simulink model "StarshipSystemModel"  (R2025b)
settings: Solver=VariableStepAuto  StartTime=0.0  StopTime=10.0  RelTol=1e-3
model workspace (MAT data in the model file):
  ActiveGNCMode : Simulink.Bus (value not decoded)
  AerodynamicControlCommand : Simulink.Bus (value not decoded)
  AerodynamicLoad : Simulink.Bus (value not decoded)
  AggregatedStream : Simulink.Bus (value not decoded)
  AllocatedEffectorDemand : Simulink.Bus (value not decoded)
  AttitudeControlDemand : Simulink.Bus (value not decoded)
  AttitudeGuidanceCommand : Simulink.Bus (value not decoded)
  AttitudeRateState : Simulink.Bus (value not decoded)
  AutogenousPressurantGas : Simulink.ConnectionBus (value not decoded)
  CandidateFaultIndication : Simulink.Bus (value not decoded)
  CombustionGasFeed : Simulink.ConnectionBus (value not decoded)
  CommandPathHealth : Simulink.Bus (value not decoded)
  ControlMode : Simulink.ValueType (value not decoded)
  DownlinkSignal : Simulink.Bus (value not decoded)
  ElectricalPower : Simulink.ConnectionBus (value not decoded)
  EngineTelemetry : Simulink.Bus (value not decoded)
  ExecutionContext : Simulink.Bus (value not decoded)
  FaultDiagnosisResult : Simulink.Bus (value not decoded)
  GNCDataContext : Simulink.Bus (value not decoded)
  GNCHealthState : Simulink.Bus (value not decoded)
  GNCStateEstimate : Simulink.Bus (value not decoded)
  GimbalAngle : Simulink.ValueType (value not decoded)
  GimbalMotion : Simulink.ConnectionBus (value not decoded)
  GroundCheckoutLink : Simulink.Bus (value not decoded)
  GroundPressurantSupply : Simulink.ConnectionBus (value not decoded)
  GuidanceConstraints : Simulink.Bus (value not decoded)
  GuidanceMode : Simulink.ValueType (value not decoded)
  LinkHealth : Simulink.Bus (value not decoded)
  LiquidPropellantFeed : Simulink.ConnectionBus (value not decoded)
  MechanicalMotion : Simulink.ConnectionBus (value not decoded)
  MechanismPosition : Simulink.Bus (value not decoded)
  ModeTransitionContext : Simulink.Bus (value not decoded)
  NavigationAidingData : Simulink.Bus (value not decoded)
  NavigationEstimate : Simulink.Bus (value not decoded)
  NavigationHealthStatus : Simulink.Bus (value not decoded)
  NavigationMeasurementSet : Simulink.Bus (value not decoded)
  PercentThrottle : Simulink.ValueType (value not decoded)
  PneumaticActuationGas : Simulink.ConnectionBus (value not decoded)
  PowerConversionStatus : Simulink.Bus (value not decoded)
  PowerDistributionStatus : Simulink.Bus (value not decoded)
  PowerHealthStatus : Simulink.Bus (value not decoded)
  PowerManagementCommand : Simulink.Bus (value not decoded)
  PowerStorageStatus : Simulink.Bus (value not decoded)
  ProtectedThermalState : Simulink.Bus (value not decoded)
  ProtectionIsolationStatus : Simulink.Bus (value not decoded)
  PurgeGasSupply : Simulink.ConnectionBus (value not decoded)
  RCSPulseCommand : Simulink.Bus (value not decoded)
  RCSTelemetry : Simulink.Bus (value not decoded)
  RFFeed : Simulink.ConnectionBus (value not decoded)
  RecoveryMechanismCommand : Simulink.Bus (value not decoded)
  RollThrottleBias : Simulink.ValueType (value not decoded)
  SafetyOverride : Simulink.ValueType (value not decoded)
  SafetyStateStatus : Simulink.Bus (value not decoded)
  ShapedControlDemand : Simulink.Bus (value not decoded)
  SpinStartIgniterGas : Simulink.ConnectionBus (value not decoded)
  StageMechanicalBoundary : Simulink.ConnectionBus (value not decoded)
  StructuralLoad : Simulink.ConnectionBus (value not decoded)
  StructureHealthStatus : Simulink.Bus (value not decoded)
  SubsystemHealthEvidence : Simulink.Bus (value not decoded)
  SubsystemStatusTelemetry : Simulink.Bus (value not decoded)
  TankTelemetry : Simulink.Bus (value not decoded)
  ThermalMonitoringCommand : Simulink.Bus (value not decoded)
  ThermalNetwork : Simulink.ConnectionBus (value not decoded)
  ThrustLoad : Simulink.ConnectionBus (value not decoded)
  TrajectoryGuidanceCommand : Simulink.Bus (value not decoded)
  TrajectoryReference : Simulink.Bus (value not decoded)
  TranslationalControlDemand : Simulink.Bus (value not decoded)
  TranslationalState : Simulink.Bus (value not decoded)
  UplinkSignal : Simulink.Bus (value not decoded)
  ValidatedControlDemand : Simulink.Bus (value not decoded)
  ValveCommand : Simulink.ValueType (value not decoded)
  VehicleStructureState : Simulink.Bus (value not decoded)
  VerifiedCommand : Simulink.Bus (value not decoded)
  VideoStream : Simulink.Bus (value not decoded)
undefined symbols (not defined in the file): ACR, ACT, ASM, ATM, BCR, BDQ, BDR, BDX, BEC, BFC, BHV, BIP, BLM, BNZ, BPI, BPR, BPV, BRX, BSM, BTA, BTP, BVC, BVE, BVV, CAA, CAM, CAS, CAT, CLM, COM, CRS, CTL, CTR, DAQ, ESC, EXT, FCR, FDB, FDE, FEX, FHI, FHM, FIC, FIS, FMG, FSC, GAP, GCM, GMD, GNC, GND, GPH, GTR, HDN, HIA, HSI, IF, INT, LOC, NAI ... (+45)
(part 5 of 8)

== system StarshipSystemModel/Starship/Safety & Fault Management /Fault Diagnosis & Isolation ==
  Bus Element In1 : Inport  PortName=IF-FDE-FCR-01
  Fault Correlation & Reasoning : Subsystem
      settings: PortSchema="{\"entries\":[{\"content\":{\"headerSize\":26,\"margin\":15,\"minimumSpacing\":25,\"sides\":[{\"content\":{\"connectorIds\":[\"In1\"]},\"type\":\"ConnectorPlacement.EquallySpacedRectSide\",\"uuid\":\"c1b9b7ae-a5d1-4a08-a561-f06fbe6dc300\"},{\"content\":{\"connectorIds\":[\"Out1\"],\"side\":\"RIGHT\"},\"type\":\"ConnectorPlacement.EquallySpacedRectSide\",\"uuid\":\"af8a3603-108a-44dc-af3d-660c23f2553a\"},{\"content\":{\"side\":\"TOP\"},\"type\":\"ConnectorPlacement.EquallySpacedRectSide\",\"uuid\":\"59101f68-40fe-4ccb-9258-ad0f93699a98\"}]},\"type\":\"ConnectorPlacement.EquallySpacedConnector\",\"uuid\":\"683df2e7-6d18-4135-a0d1-7e7a3e3475d2\"}],\"packageUris\":[\"http://schema.mathworks.com/mf0/Connector/R2020b\"],\"version\":\"1.0\"}"
  Fault Identification & Classification : Subsystem
      settings: PortSchema="{\"entries\":[{\"content\":{\"headerSize\":26,\"margin\":15,\"minimumSpacing\":25,\"sides\":[{\"content\":{\"connectorIds\":[\"In1\"]},\"type\":\"ConnectorPlacement.EquallySpacedRectSide\",\"uuid\":\"c1b9b7ae-a5d1-4a08-a561-f06fbe6dc300\"},{\"content\":{\"connectorIds\":[\"Out1\"],\"side\":\"RIGHT\"},\"type\":\"ConnectorPlacement.EquallySpacedRectSide\",\"uuid\":\"af8a3603-108a-44dc-af3d-660c23f2553a\"},{\"content\":{\"side\":\"TOP\"},\"type\":\"ConnectorPlacement.EquallySpacedRectSide\",\"uuid\":\"59101f68-40fe-4ccb-9258-ad0f93699a98\"}]},\"type\":\"ConnectorPlacement.EquallySpacedConnector\",\"uuid\":\"683df2e7-6d18-4135-a0d1-7e7a3e3475d2\"}],\"packageUris\":[\"http://schema.mathworks.com/mf0/Connector/R2020b\"],\"version\":\"1.0\"}"
  Fault Isolation : Subsystem
      settings: PortSchema="{\"entries\":[{\"content\":{\"headerSize\":26,\"margin\":15,\"minimumSpacing\":25,\"sides\":[{\"content\":{\"connectorIds\":[\"In1\"]},\"type\":\"ConnectorPlacement.EquallySpacedRectSide\",\"uuid\":\"c1b9b7ae-a5d1-4a08-a561-f06fbe6dc300\"},{\"content\":{\"connectorIds\":[\"Out1\"],\"side\":\"RIGHT\"},\"type\":\"ConnectorPlacement.EquallySpacedRectSide\",\"uuid\":\"af8a3603-108a-44dc-af3d-660c23f2553a\"},{\"content\":{\"side\":\"TOP\"},\"type\":\"ConnectorPlacement.EquallySpacedRectSide\",\"uuid\":\"59101f68-40fe-4ccb-9258-ad0f93699a98\"}]},\"type\":\"ConnectorPlacement.EquallySpacedConnector\",\"uuid\":\"683df2e7-6d18-4135-a0d1-7e7a3e3475d2\"}],\"packageUris\":[\"http://schema.mathworks.com/mf0/Connector/R2020b\"],\"version\":\"1.0\"}"
  Bus Element Out1 : Outport  PortName=IF-FIC-SEA-01
  wires:
  Fault Isolation/1(IF-FIS-FIC-01) -> Fault Identification & Classification/1(IF-FIS-FIC-01)
  Bus Element In1/1 -> Fault Correlation & Reasoning/1(IF-FDE-FCR-01)
  Fault Correlation & Reasoning/1(IF-FCR-FIS-01) -> Fault Isolation/1(IF-FCR-FIS-01)
  Fault Identification & Classification/1(IF-FIC-SEA-01) -> Bus Element Out1/1

== system StarshipSystemModel/Starship/Safety & Fault Management /Fault Management & Response Logic ==
  Bus Element In1 : Inport  PortName=IF-FIC-SEA-01
  Protective Action Coordination : Subsystem
      settings: PortSchema="{\"entries\":[{\"content\":{\"headerSize\":26,\"margin\":15,\"minimumSpacing\":25,\"sides\":[{\"content\":{\"connectorIds\":[\"In1\"]},\"type\":\"ConnectorPlacement.EquallySpacedRectSide\",\"uuid\":\"c1b9b7ae-a5d1-4a08-a561-f06fbe6dc300\"},{\"content\":{\"connectorIds\":[\"Out1\",\"Out2\",\"Out3\"],\"side\":\"RIGHT\"},\"type\":\"ConnectorPlacement.EquallySpacedRectSide\",\"uuid\":\"af8a3603-108a-44dc-af3d-660c23f2553a\"},{\"content\":{\"side\":\"TOP\"},\"type\":\"ConnectorPlacement.EquallySpacedRectSide\",\"uuid\":\"59101f68-40fe-4ccb-9258-ad0f93699a98\"}]},\"type\":\"ConnectorPlacement.EquallySpacedConnector\",\"uuid\":\"683df2e7-6d18-4135-a0d1-7e7a3e3475d2\"}],\"packageUris\":[\"http://schema.mathworks.com/mf0/Connector/R2020b\"],\"version\":\"1.0\"}"
  Response Selection Logic : Subsystem
      settings: PortSchema="{\"entries\":[{\"content\":{\"headerSize\":26,\"margin\":15,\"minimumSpacing\":25,\"sides\":[{\"content\":{\"connectorIds\":[\"In1\"]},\"type\":\"ConnectorPlacement.EquallySpacedRectSide\",\"uuid\":\"c1b9b7ae-a5d1-4a08-a561-f06fbe6dc300\"},{\"content\":{\"connectorIds\":[\"Out1\"],\"side\":\"RIGHT\"},\"type\":\"ConnectorPlacement.EquallySpacedRectSide\",\"uuid\":\"af8a3603-108a-44dc-af3d-660c23f2553a\"},{\"content\":{\"side\":\"TOP\"},\"type\":\"ConnectorPlacement.EquallySpacedRectSide\",\"uuid\":\"59101f68-40fe-4ccb-9258-ad0f93699a98\"}]},\"type\":\"ConnectorPlacement.EquallySpacedConnector\",\"uuid\":\"683df2e7-6d18-4135-a0d1-7e7a3e3475d2\"}],\"packageUris\":[\"http://schema.mathworks.com/mf0/Connector/R2020b\"],\"version\":\"1.0\"}"
  Severity & Consequence Assessment : Subsystem
      settings: PortSchema="{\"entries\":[{\"content\":{\"headerSize\":26,\"margin\":15,\"minimumSpacing\":25,\"sides\":[{\"content\":{\"connectorIds\":[\"In1\"]},\"type\":\"ConnectorPlacement.EquallySpacedRectSide\",\"uuid\":\"c1b9b7ae-a5d1-4a08-a561-f06fbe6dc300\"},{\"content\":{\"connectorIds\":[\"Out1\"],\"side\":\"RIGHT\"},\"type\":\"ConnectorPlacement.EquallySpacedRectSide\",\"uuid\":\"af8a3603-108a-44dc-af3d-660c23f2553a\"},{\"content\":{\"side\":\"TOP\"},\"type\":\"ConnectorPlacement.EquallySpacedRectSide\",\"uuid\":\"59101f68-40fe-4ccb-9258-ad0f93699a98\"}]},\"type\":\"ConnectorPlacement.EquallySpacedConnector\",\"uuid\":\"683df2e7-6d18-4135-a0d1-7e7a3e3475d2\"}],\"packageUris\":[\"http://schema.mathworks.com/mf0/Connector/R2020b\"],\"version\":\"1.0\"}"
  Bus Element Out1 : Outport  PortName=IF-SAF-BEC-01
  Bus Element Out2 : Outport  Port=2  PortName=IF-SAF-SEC-01
  Bus Element Out3 : Outport  Port=3  PortName=IF-PAC-RCO-01
  wires:
  Protective Action Coordination/2(IF-SAF-SEC-01) -> Bus Element Out2/1
  Response Selection Logic/1(IF-RSL-PAC-01) -> Protective Action Coordination/1(IF-RSL-PAC-01)
  Bus Element In1/1 -> Severity & Consequence Assessment/1(IF-FIC-SEA-01)
  Severity & Consequence Assessment/1(IF-SEA-RSL-01) -> Response Selection Logic/1(IF-SEA-RSL-01)
  Protective Action Coordination/3(IF-PAC-RCO-01) -> Bus Element Out3/1
  Protective Action Coordination/1(IF-SAF-BEC-01) -> Bus Element Out1/1

== system StarshipSystemModel/Starship/Safety & Fault Management /Health Monitoring & Fault Detection ==
  Bus Element In11 : Inport  PortName=IF-RSM-SAF-01
  Bus Element In10 : Inport  Port=2  PortName=IF-INT-SAF-01
  Bus Element In9 : Inport  Port=3  PortName=IF-POS-SAF-01
  Bus Element In8 : Inport  Port=4  PortName=IF-TMS-SAF-01
  Bus Element In7 : Inport  Port=5  PortName=IF-FHM-SAF-01
  Bus Element In1 : Inport  Port=6  PortName=IF-BEC-SAF-01
  Bus Element In2 : Inport  Port=7  PortName=IF-SEC-SAF-01
  Bus Element In3 : Inport  Port=8  PortName=IF-RCT-SAF-01
  Bus Element In4 : Inport  Port=9  PortName=IF-BPR-SAF-01
  Bus Element In5 : Inport  Port=10  PortName=IF-SPR-SAF-01
  Bus Element In6 : Inport  Port=11  PortName=IF-PMM-SAF-01
  Bus Element In12 : Inport  Port=12  PortName=IF-BLM-SAF-01
  Bus Element In13 : Inport  Port=13  PortName=IF-SLM-SAF-01
  Bus Element In14 : Inport  Port=14  PortName=IF-ESC-HIA-01
  Fault Detection Engine : Subsystem
      settings: PortSchema="{\"entries\":[{\"content\":{\"headerSize\":26,\"margin\":15,\"minimumSpacing\":25,\"sides\":[{\"content\":{\"connectorIds\":[\"In1\"]},\"type\":\"ConnectorPlacement.EquallySpacedRectSide\",\"uuid\":\"c1b9b7ae-a5d1-4a08-a561-f06fbe6dc300\"},{\"content\":{\"connectorIds\":[\"Out1\"],\"side\":\"RIGHT\"},\"type\":\"ConnectorPlacement.EquallySpacedRectSide\",\"uuid\":\"af8a3603-108a-44dc-af3d-660c23f2553a\"},{\"content\":{\"side\":\"TOP\"},\"type\":\"ConnectorPlacement.EquallySpacedRectSide\",\"uuid\":\"59101f68-40fe-4ccb-9258-ad0f93699a98\"}]},\"type\":\"ConnectorPlacement.EquallySpacedConnector\",\"uuid\":\"683df2e7-6d18-4135-a0d1-7e7a3e3475d2\"}],\"packageUris\":[\"http://schema.mathworks.com/mf0/Connector/R2020b\"],\"version\":\"1.0\"}"
  Health Information Aggregation : Subsystem
      settings: PortSchema="{\"entries\":[{\"content\":{\"headerSize\":26,\"margin\":15,\"minimumSpacing\":25,\"sides\":[{\"content\":{\"connectorIds\":[\"In1\",\"In2\",\"In3\",\"In4\",\"In5\",\"In6\",\"In7\",\"In8\",\"In9\",\"In10\",\"In11\",\"In12\",\"In13\",\"In14\"]},\"type\":\"ConnectorPlacement.EquallySpacedRectSide\",\"uuid\":\"c1b9b7ae-a5d1-4a08-a561-f06fbe6dc300\"},{\"content\":{\"connectorIds\":[\"Out1\"],\"side\":\"RIGHT\"},\"type\":\"ConnectorPlacement.EquallySpacedRectSide\",\"uuid\":\"af8a3603-108a-44dc-af3d-660c23f2553a\"},{\"content\":{\"side\":\"TOP\"},\"type\":\"ConnectorPlacement.EquallySpacedRectSide\",\"uuid\":\"59101f68-40fe-4ccb-9258-ad0f93699a98\"}]},\"type\":\"ConnectorPlacement.EquallySpacedConnector\",\"uuid\":\"683df2e7-6d18-4135-a0d1-7e7a3e3475d2\"}],\"packageUris\":[\"http://schema.mathworks.com/mf0/Connector/R2020b\"],\"version\":\"1.0\"}"
  Validity & Integrity Evaluation : Subsystem
      settings: PortSchema="{\"entries\":[{\"content\":{\"headerSize\":26,\"margin\":15,\"minimumSpacing\":25,\"sides\":[{\"content\":{\"connectorIds\":[\"In1\"]},\"type\":\"ConnectorPlacement.EquallySpacedRectSide\",\"uuid\":\"c1b9b7ae-a5d1-4a08-a561-f06fbe6dc300\"},{\"content\":{\"connectorIds\":[\"Out1\"],\"side\":\"RIGHT\"},\"type\":\"ConnectorPlacement.EquallySpacedRectSide\",\"uuid\":\"af8a3603-108a-44dc-af3d-660c23f2553a\"},{\"content\":{\"side\":\"TOP\"},\"type\":\"ConnectorPlacement.EquallySpacedRectSide\",\"uuid\":\"59101f68-40fe-4ccb-9258-ad0f93699a98\"}]},\"type\":\"ConnectorPlacement.EquallySpacedConnector\",\"uuid\":\"683df2e7-6d18-4135-a0d1-7e7a3e3475d2\"}],\"packageUris\":[\"http://schema.mathworks.com/mf0/Connector/R2020b\"],\"version\":\"1.0\"}"
  Bus Element Out1 : Outport  PortName=IF-FDE-FCR-01
  wires:
  Bus Element In11/1 -> Health Information Aggregation/1(IF-RSM-SAF-01)
  Bus Element In10/1 -> Health Information Aggregation/2(IF-INT-SAF-01)
  Bus Element In3/1 -> Health Information Aggregation/8(IF-RCT-SAF-01)
  Bus Element In2/1 -> Health Information Aggregation/7(IF-SEC-SAF-01)
  Bus Element In1/1 -> Health Information Aggregation/6(IF-BEC-SAF-01)
  Bus Element In9/1 -> Health Information Aggregation/3(IF-POS-SAF-01)
  Bus Element In7/1 -> Health Information Aggregation/5(IF-FHM-SAF-01)
  Bus Element In8/1 -> Health Information Aggregation/4(IF-TMS-SAF-01)
  Bus Element In4/1 -> Health Information Aggregation/9(IF-BPR-SAF-01)
  Bus Element In5/1 -> Health Information Aggregation/10(IF-SPR-SAF-01)
  Bus Element In6/1 -> Health Information Aggregation/11(IF-PMM-SAF-01)
  Validity & Integrity Evaluation/1(IF-VIE-FDE-01) -> Fault Detection Engine/1(IF-VIE-FDE-01)
  Bus Element In12/1 -> Health Information Aggregation/12(IF-BLM-SAF-01)
  Bus Element In13/1 -> Health Information Aggregation/13(IF-SLM-SAF-01)
  Bus Element In14/1 -> Health Information Aggregation/14(IF-ESC-HIA-01)
  Health Information Aggregation/1(IF-HIA-VIE-01) -> Validity & Integrity Evaluation/1(IF-HIA-VIE-01)
  Fault Detection Engine/1(IF-FDE-FCR-01) -> Bus Element Out1/1

== system StarshipSystemModel/Starship/Safety & Fault Management /Recovery & Reconfiguration Management ==
  Bus Element In1 : Inport  PortName=IF-PAC-RCO-01
  Reconfiguration Coordinator : Subsystem
      settings: PortSchema="{\"entries\":[{\"content\":{\"headerSize\":26,\"margin\":15,\"minimumSpacing\":25,\"sides\":[{\"content\":{\"connectorIds\":[\"In1\"]},\"type\":\"ConnectorPlacement.EquallySpacedRectSide\",\"uuid\":\"c1b9b7ae-a5d1-4a08-a561-f06fbe6dc300\"},{\"content\":{\"connectorIds\":[\"Out1\"],\"side\":\"RIGHT\"},\"type\":\"ConnectorPlacement.EquallySpacedRectSide\",\"uuid\":\"af8a3603-108a-44dc-af3d-660c23f2553a\"},{\"content\":{\"side\":\"TOP\"},\"type\":\"ConnectorPlacement.EquallySpacedRectSide\",\"uuid\":\"59101f68-40fe-4ccb-9258-ad0f93699a98\"}]},\"type\":\"ConnectorPlacement.EquallySpacedConnector\",\"uuid\":\"683df2e7-6d18-4135-a0d1-7e7a3e3475d2\"}],\"packageUris\":[\"http://schema.mathworks.com/mf0/Connector/R2020b\"],\"version\":\"1.0\"}"
  Recovery Sequence Executor : Subsystem
      settings: PortSchema="{\"entries\":[{\"content\":{\"headerSize\":26,\"margin\":15,\"minimumSpacing\":25,\"sides\":[{\"content\":{\"connectorIds\":[\"In1\"]},\"type\":\"ConnectorPlacement.EquallySpacedRectSide\",\"uuid\":\"c1b9b7ae-a5d1-4a08-a561-f06fbe6dc300\"},{\"content\":{\"connectorIds\":[\"Out1\",\"Out2\"],\"side\":\"RIGHT\"},\"type\":\"ConnectorPlacement.EquallySpacedRectSide\",\"uuid\":\"af8a3603-108a-44dc-af3d-660c23f2553a\"},{\"content\":{\"side\":\"TOP\"},\"type\":\"ConnectorPlacement.EquallySpacedRectSide\",\"uuid\":\"59101f68-40fe-4ccb-9258-ad0f93699a98\"}]},\"type\":\"ConnectorPlacement.EquallySpacedConnector\",\"uuid\":\"683df2e7-6d18-4135-a0d1-7e7a3e3475d2\"}],\"packageUris\":[\"http://schema.mathworks.com/mf0/Connector/R2020b\"],\"version\":\"1.0\"}"
  Recovery Verification : Subsystem
      settings: PortSchema="{\"entries\":[{\"content\":{\"headerSize\":26,\"margin\":15,\"minimumSpacing\":25,\"sides\":[{\"content\":{\"connectorIds\":[\"In1\"]},\"type\":\"ConnectorPlacement.EquallySpacedRectSide\",\"uuid\":\"c1b9b7ae-a5d1-4a08-a561-f06fbe6dc300\"},{\"content\":{\"connectorIds\":[\"Out1\"],\"side\":\"RIGHT\"},\"type\":\"ConnectorPlacement.EquallySpacedRectSide\",\"uuid\":\"af8a3603-108a-44dc-af3d-660c23f2553a\"},{\"content\":{\"side\":\"TOP\"},\"type\":\"ConnectorPlacement.EquallySpacedRectSide\",\"uuid\":\"59101f68-40fe-4ccb-9258-ad0f93699a98\"}]},\"type\":\"ConnectorPlacement.EquallySpacedConnector\",\"uuid\":\"683df2e7-6d18-4135-a0d1-7e7a3e3475d2\"}],\"packageUris\":[\"http://schema.mathworks.com/mf0/Connector/R2020b\"],\"version\":\"1.0\"}"
  Bus Element Out1 : Outport  PortName=IF-SAF-RSM-01
  Bus Element Out2 : Outport  Port=2  PortName=IF-RVF-SSM-01
  wires:
  Recovery Sequence Executor/2(IF-RSE-RVF-01) -> Recovery Verification/1(IF-RSE-RVF-01)
  Bus Element In1/1 -> Reconfiguration Coordinator/1(IF-PAC-RCO-01)
  Reconfiguration Coordinator/1(IF-RCO-RSE-01) -> Recovery Sequence Executor/1(IF-RCO-RSE-01)
  Recovery Sequence Executor/1(IF-SAF-RSM-01) -> Bus Element Out1/1
  Recovery Verification/1(IF-RVF-SSM-01) -> Bus Element Out2/1

== system StarshipSystemModel/Starship/Safety & Fault Management /Safety State & Flight-Safety Management ==
  Bus Element In3 : Inport  PortName=IF-RVF-SSM-01
  Bus Element In1 : Inport  Port=2  PortName=IF-BCR-SAF-01
  Bus Element In2 : Inport  Port=3  PortName=IF-SCR-SAF-01
  Escalation & Containment Status : Subsystem
      settings: PortSchema="{\"entries\":[{\"content\":{\"headerSize\":26,\"margin\":15,\"minimumSpacing\":25,\"sides\":[{\"content\":{\"connectorIds\":[\"In1\"]},\"type\":\"ConnectorPlacement.EquallySpacedRectSide\",\"uuid\":\"c1b9b7ae-a5d1-4a08-a561-f06fbe6dc300\"},{\"content\":{\"connectorIds\":[\"Out2\",\"Out1\",\"Out3\"],\"side\":\"RIGHT\"},\"type\":\"ConnectorPlacement.EquallySpacedRectSide\",\"uuid\":\"af8a3603-108a-44dc-af3d-660c23f2553a\"},{\"content\":{\"side\":\"TOP\"},\"type\":\"ConnectorPlacement.EquallySpacedRectSide\",\"uuid\":\"59101f68-40fe-4ccb-9258-ad0f93699a98\"},{\"content\":{\"side\":\"BOTTOM\"},\"type\":\"ConnectorPlacement.EquallySpacedRectSide\",\"uuid\":\"baebb347-8adb-49bd-9e46-495e8e474d7d\"}]},\"type\":\"ConnectorPlacement.EquallySpacedConnector\",\"uuid\":\"683df2e7-6d18-4135-a0d1-7e7a3e3475d2\"}],\"packageUris\":[\"http://schema.mathworks.com/mf0/Connector/R2020b\"],\"version\":\"1.0\"}"
  Flight-Safety Coordination : Subsystem
      settings: PortSchema="{\"entries\":[{\"content\":{\"headerSize\":26,\"margin\":15,\"minimumSpacing\":25,\"sides\":[{\"content\":{\"connectorIds\":[\"In1\",\"In2\",\"In3\"]},\"type\":\"ConnectorPlacement.EquallySpacedRectSide\",\"uuid\":\"c1b9b7ae-a5d1-4a08-a561-f06fbe6dc300\"},{\"content\":{\"connectorIds\":[\"Out1\"],\"side\":\"RIGHT\"},\"type\":\"ConnectorPlacement.EquallySpacedRectSide\",\"uuid\":\"af8a3603-108a-44dc-af3d-660c23f2553a\"},{\"content\":{\"side\":\"TOP\"},\"type\":\"ConnectorPlacement.EquallySpacedRectSide\",\"uuid\":\"59101f68-40fe-4ccb-9258-ad0f93699a98\"}]},\"type\":\"ConnectorPlacement.EquallySpacedConnector\",\"uuid\":\"683df2e7-6d18-4135-a0d1-7e7a3e3475d2\"}],\"packageUris\":[\"http://schema.mathworks.com/mf0/Connector/R2020b\"],\"version\":\"1.0\"}"
  Safety State Manager : Subsystem
      settings: PortSchema="{\"entries\":[{\"content\":{\"headerSize\":26,\"margin\":15,\"minimumSpacing\":25,\"sides\":[{\"content\":{\"connectorIds\":[\"In1\"]},\"type\":\"ConnectorPlacement.EquallySpacedRectSide\",\"uuid\":\"c1b9b7ae-a5d1-4a08-a561-f06fbe6dc300\"},{\"content\":{\"connectorIds\":[\"Out1\",\"Out2\"],\"side\":\"RIGHT\"},\"type\":\"ConnectorPlacement.EquallySpacedRectSide\",\"uuid\":\"af8a3603-108a-44dc-af3d-660c23f2553a\"},{\"content\":{\"side\":\"TOP\"},\"type\":\"ConnectorPlacement.EquallySpacedRectSide\",\"uuid\":\"59101f68-40fe-4ccb-9258-ad0f93699a98\"}]},\"type\":\"ConnectorPlacement.EquallySpacedConnector\",\"uuid\":\"683df2e7-6d18-4135-a0d1-7e7a3e3475d2\"}],\"packageUris\":[\"http://schema.mathworks.com/mf0/Connector/R2020b\"],\"version\":\"1.0\"}"
  Bus Element Out2 : Outport  PortName=IF-SAF-BTA-01
  Bus Element Out3 : Outport  Port=2  PortName=IF-SAF-STA-01
  Bus Element Out1 : Outport  Port=3  PortName=IF-SAF-FHM-01
  Bus Element Out4 : Outport  Port=4  PortName=IF-ESC-HIA-01
  wires:
  Flight-Safety Coordination/1(IF-FSC-ESC-01) -> Escalation & Containment Status/1(IF-FSC-ESC-01)
  Bus Element In3/1 -> Safety State Manager/1(IF-RVF-SSM-01)
  Safety State Manager/2(IF-SSM-FSC-01) -> Flight-Safety Coordination/3(IF-SSM-FSC-01)
  Escalation & Containment Status/2(IF-SAF-BTA-01) -> Bus Element Out2/1
  Bus Element In1/1 -> Flight-Safety Coordination/1(IF-BCR-SAF-01)
  Bus Element In2/1 -> Flight-Safety Coordination/2(IF-SCR-SAF-01)
  Safety State Manager/1(IF-SAF-FHM-01) -> Bus Element Out1/1
  Escalation & Containment Status/1(IF-SAF-STA-01) -> Bus Element Out3/1
  Escalation & Containment Status/3(IF-ESC-HIA-01) -> Bus Element Out4/1

== system StarshipSystemModel/Starship/Structure and Mechanisms/Aerodynamic Control Mechanisms ==
  Bus Element In1 : Inport  PortName=IF-GNC-ACT-01
  Bus Element In2 : Inport  Port=2  PortName=IF-ATM-SUR-01
  Actuator : Subsystem
      settings: PortSchema="{\"entries\":[{\"content\":{\"headerSize\":26,\"margin\":15,\"minimumSpacing\":25,\"sides\":[{\"content\":{\"connectorIds\":[\"In1\",\"In2\",\"LConn1\"]},\"type\":\"ConnectorPlacement.EquallySpacedRectSide\",\"uuid\":\"23792f18-2863-4199-9730-8799d4a474a5\"},{\"content\":{\"connectorIds\":[\"RConn1\"],\"side\":\"RIGHT\"},\"type\":\"ConnectorPlacement.EquallySpacedRectSide\",\"uuid\":\"c8cda51b-7b41-45d2-a922-70343296893f\"},{\"content\":{\"side\":\"TOP\"},\"type\":\"ConnectorPlacement.EquallySpacedRectSide\",\"uuid\":\"3580f4a1-1924-4d7f-ad03-70e3a97c03ce\"}]},\"type\":\"ConnectorPlacement.EquallySpacedConnector\",\"uuid\":\"f1529067-176f-4d7b-82ef-d3d6162373fd\"}],\"packageUris\":[\"http://schema.mathworks.com/mf0/Connector/R2020b\"],\"version\":\"1.0\"}"
  Hinge / linkage : Subsystem
      settings: PortSchema="{\"entries\":[{\"content\":{\"headerSize\":26,\"margin\":15,\"minimumSpacing\":25,\"sides\":[{\"content\":{\"connectorIds\":[\"LConn1\",\"LConn2\"]},\"type\":\"ConnectorPlacement.EquallySpacedRectSide\",\"uuid\":\"23792f18-2863-4199-9730-8799d4a474a5\"},{\"content\":{\"connectorIds\":[\"RConn1\",\"RConn2\"],\"side\":\"RIGHT\"},\"type\":\"ConnectorPlacement.EquallySpacedRectSide\",\"uuid\":\"c8cda51b-7b41-45d2-a922-70343296893f\"},{\"content\":{\"side\":\"TOP\"},\"type\":\"ConnectorPlacement.EquallySpacedRectSide\",\"uuid\":\"3580f4a1-1924-4d7f-ad03-70e3a97c03ce\"}]},\"type\":\"ConnectorPlacement.EquallySpacedConnector\",\"uuid\":\"f1529067-176f-4d7b-82ef-d3d6162373fd\"}],\"packageUris\":[\"http://schema.mathworks.com/mf0/Connector/R2020b\"],\"version\":\"1.0\"}"
  Position / health : Subsystem
      settings: PortSchema="{\"entries\":[{\"content\":{\"headerSize\":26,\"margin\":15,\"minimumSpacing\":25,\"sides\":[{\"content\":{},\"type\":\"ConnectorPlacement.EquallySpacedRectSide\",\"uuid\":\"23792f18-2863-4199-9730-8799d4a474a5\"},{\"content\":{\"connectorIds\":[\"Out1\",\"Out2\",\"Out3\"],\"side\":\"RIGHT\"},\"type\":\"ConnectorPlacement.EquallySpacedRectSide\",\"uuid\":\"c8cda51b-7b41-45d2-a922-70343296893f\"},{\"content\":{\"side\":\"TOP\"},\"type\":\"ConnectorPlacement.EquallySpacedRectSide\",\"uuid\":\"3580f4a1-1924-4d7f-ad03-70e3a97c03ce\"}]},\"type\":\"ConnectorPlacement.EquallySpacedConnector\",\"uuid\":\"f1529067-176f-4d7b-82ef-d3d6162373fd\"}],\"packageUris\":[\"http://schema.mathworks.com/mf0/Connector/R2020b\"],\"version\":\"1.0\"}"
  Surface / fin / flap : Subsystem
      settings: PortSchema="{\"entries\":[{\"content\":{\"headerSize\":26,\"margin\":15,\"minimumSpacing\":25,\"sides\":[{\"content\":{\"connectorIds\":[\"In1\",\"LConn1\"]},\"type\":\"ConnectorPlacement.EquallySpacedRectSide\",\"uuid\":\"23792f18-2863-4199-9730-8799d4a474a5\"},{\"content\":{\"connectorIds\":[\"RConn1\"],\"side\":\"RIGHT\"},\"type\":\"ConnectorPlacement.EquallySpacedRectSide\",\"uuid\":\"c8cda51b-7b41-45d2-a922-70343296893f\"},{\"content\":{\"side\":\"TOP\"},\"type\":\"ConnectorPlacement.EquallySpacedRectSide\",\"uuid\":\"3580f4a1-1924-4d7f-ad03-70e3a97c03ce\"}]},\"type\":\"ConnectorPlacement.EquallySpacedConnector\",\"uuid\":\"f1529067-176f-4d7b-82ef-d3d6162373fd\"}],\"packageUris\":[\"http://schema.mathworks.com/mf0/Connector/R2020b\"],\"version\":\"1.0\"}"
  IF-HNG-INT-01 : PMIOPort  Side=Right
  IF-PWR-STR-01 : PMIOPort  Port=2  Side=Left  ConnectionType=Bus: ElectricalPower
  Bus Element Out1 : Outport  PortName=IF-POS-GNC-01
  Bus Element Out2 : Outport  Port=2  PortName=IF-POS-SAF-01
  wires:
  Position / health/1(IF-POS-GNC-01) -> Bus Element Out1/1
  Position / health/2(IF-POS-ACT-01) -> Actuator/2(IF-POS-ACT-01)
  Bus Element In1/1 -> Actuator/1(IF-GNC-ACT-01)
  Bus Element In2/1 -> Surface / fin / flap/1(IF-ATM-SUR-01)
  Position / health/3(IF-POS-SAF-01) -> Bus Element Out2/1
  connections:
  Hinge / linkage/RConn2 -- IF-HNG-INT-01/RConn1
  Actuator/RConn1 -- Hinge / linkage/LConn2
  Hinge / linkage/RConn1 -- Surface / fin / flap/LConn1
  Surface / fin / flap/RConn1 -- Hinge / linkage/LConn1
  IF-PWR-STR-01/RConn1 -- Actuator/LConn1

== system StarshipSystemModel/Starship/Structure and Mechanisms/Primary Load-Bearing Airframe ==
  " Load-transfer structure" : Subsystem
      settings: PortSchema="{\"entries\":[{\"content\":{\"headerSize\":26,\"margin\":15,\"minimumSpacing\":25,\"sides\":[{\"content\":{\"connectorIds\":[\"LConn1\",\"LConn2\"]},\"type\":\"ConnectorPlacement.EquallySpacedRectSide\",\"uuid\":\"23792f18-2863-4199-9730-8799d4a474a5\"},{\"content\":{\"connectorIds\":[\"RConn1\"],\"side\":\"RIGHT\"},\"type\":\"ConnectorPlacement.EquallySpacedRectSide\",\"uuid\":\"c8cda51b-7b41-45d2-a922-70343296893f\"},{\"content\":{\"side\":\"TOP\"},\"type\":\"ConnectorPlacement.EquallySpacedRectSide\",\"uuid\":\"3580f4a1-1924-4d7f-ad03-70e3a97c03ce\"}]},\"type\":\"ConnectorPlacement.EquallySpacedConnector\",\"uuid\":\"f1529067-176f-4d7b-82ef-d3d6162373fd\"}],\"packageUris\":[\"http://schema.mathworks.com/mf0/Connector/R2020b\"],\"version\":\"1.0\"}"
  Local interface structure : Subsystem
      settings: PortSchema="{\"entries\":[{\"content\":{\"headerSize\":26,\"margin\":15,\"minimumSpacing\":25,\"sides\":[{\"content\":{\"connectorIds\":[\"LConn1\",\"LConn2\",\"LConn3\"]},\"type\":\"ConnectorPlacement.EquallySpacedRectSide\",\"uuid\":\"23792f18-2863-4199-9730-8799d4a474a5\"},{\"content\":{\"connectorIds\":[\"Out1\",\"Out2\",\"Out3\",\"RConn1\"],\"side\":\"RIGHT\"},\"type\":\"ConnectorPlacement.EquallySpacedRectSide\",\"uuid\":\"c8cda51b-7b41-45d2-a922-70343296893f\"},{\"content\":{\"side\":\"TOP\"},\"type\":\"ConnectorPlacement.EquallySpacedRectSide\",\"uuid\":\"3580f4a1-1924-4d7f-ad03-70e3a97c03ce\"}]},\"type\":\"ConnectorPlacement.EquallySpacedConnector\",\"uuid\":\"f1529067-176f-4d7b-82ef-d3d6162373fd\"}],\"packageUris\":[\"http://schema.mathworks.com/mf0/Connector/R2020b\"],\"version\":\"1.0\"}"
  Primary pressure/shell : Subsystem
      settings: PortSchema="{\"entries\":[{\"content\":{\"headerSize\":26,\"margin\":15,\"minimumSpacing\":25,\"sides\":[{\"content\":{\"connectorIds\":[\"RConn2\",\"RConn1\",\"LConn1\",\"LConn2\",\"LConn3\",\"LConn4\",\"LConn5\"]},\"type\":\"ConnectorPlacement.EquallySpacedRectSide\",\"uuid\":\"23792f18-2863-4199-9730-8799d4a474a5\"},{\"content\":{\"connectorIds\":[\"RConn3\"],\"side\":\"RIGHT\"},\"type\":\"ConnectorPlacement.EquallySpacedRectSide\",\"uuid\":\"c8cda51b-7b41-45d2-a922-70343296893f\"},{\"content\":{\"side\":\"TOP\"},\"type\":\"ConnectorPlacement.EquallySpacedRectSide\",\"uuid\":\"3580f4a1-1924-4d7f-ad03-70e3a97c03ce\"}]},\"type\":\"ConnectorPlacement.EquallySpacedConnector\",\"uuid\":\"f1529067-176f-4d7b-82ef-d3d6162373fd\"}],\"packageUris\":[\"http://schema.mathworks.com/mf0/Connector/R2020b\"],\"version\":\"1.0\"}"
  IF-TLI-LDT-01 : PMIOPort  Side=Right
  IF-BOT-PRS-01 : PMIOPort  Port=2  Side=Right  ConnectionType=Bus: StructuralLoad
  IF-SOT-PRS-01 : PMIOPort  Port=3  Side=Right  ConnectionType=Bus: StructuralLoad
  IF-TBI-PRS-01 : PMIOPort  Port=4  Side=Left  ConnectionType=Bus: ThermalNetwork
  IF-BTP-PRS-01 : PMIOPort  Port=5  Side=Left  ConnectionType=Bus: ThermalNetwork
  IF-STP-PRS-01 : PMIOPort  Port=6  Side=Left  ConnectionType=Bus: ThermalNetwork
  IF-HNG-INT-01 : PMIOPort  Port=7  Side=Left
  IF-SLS-LDT-01 : PMIOPort  Port=8  Side=Left
  IF-RLI-PRS-01 : PMIOPort  Port=9  Side=Left
  Bus Element Out1 : Outport  PortName=IF-INT-STA-01
  Bus Element Out2 : Outport  Port=2  PortName=IF-INT-BTA-01
  Bus Element Out3 : Outport  Port=3  PortName=IF-INT-SAF-01
  wires:
  Local interface structure/2(IF-INT-STA-01) -> Bus Element Out1/1
  Local interface structure/3(IF-INT-BTA-01) -> Bus Element Out2/1
  Local interface structure/1(IF-INT-SAF-01) -> Bus Element Out3/1
  connections:
  IF-RLI-PRS-01/RConn1 -- Primary pressure/shell/LConn1
  Primary pressure/shell/RConn1 -- IF-BOT-PRS-01/RConn1
  IF-TBI-PRS-01/RConn1 -- Primary pressure/shell/LConn2
  Primary pressure/shell/RConn2 -- IF-SOT-PRS-01/RConn1
  IF-BTP-PRS-01/RConn1 -- Primary pressure/shell/LConn3
  IF-STP-PRS-01/RConn1 -- Primary pressure/shell/LConn4
  IF-TLI-LDT-01/RConn1 -- " Load-transfer structure"/LConn2
  Primary pressure/shell/RConn3 -- " Load-transfer structure"/LConn1
  " Load-transfer structure"/RConn1 -- Local interface structure/LConn1
  IF-SLS-LDT-01/RConn1 -- Local interface structure/LConn2
  IF-HNG-INT-01/RConn1 -- Local interface structure/LConn3
  Local interface structure/RConn1 -- Primary pressure/shell/LConn5

== system StarshipSystemModel/Starship/Structure and Mechanisms/Recovery & Landing Mechanisms ==
  Bus Element In1 : Inport  PortName=IF-SAF-RSM-01
  Landing/catch load path : Subsystem
      settings: PortSchema="{\"entries\":[{\"content\":{\"headerSize\":26,\"margin\":15,\"minimumSpacing\":25,\"sides\":[{\"content\":{\"connectorIds\":[\"LConn1\"]},\"type\":\"ConnectorPlacement.EquallySpacedRectSide\",\"uuid\":\"23792f18-2863-4199-9730-8799d4a474a5\"},{\"content\":{\"connectorIds\":[\"RConn1\",\"RConn2\"],\"side\":\"RIGHT\"},\"type\":\"ConnectorPlacement.EquallySpacedRectSide\",\"uuid\":\"c8cda51b-7b41-45d2-a922-70343296893f\"},{\"content\":{\"side\":\"TOP\"},\"type\":\"ConnectorPlacement.EquallySpacedRectSide\",\"uuid\":\"3580f4a1-1924-4d7f-ad03-70e3a97c03ce\"}]},\"type\":\"ConnectorPlacement.EquallySpacedConnector\",\"uuid\":\"f1529067-176f-4d7b-82ef-d3d6162373fd\"}],\"packageUris\":[\"http://schema.mathworks.com/mf0/Connector/R2020b\"],\"version\":\"1.0\"}"
  Recovery mechanism : Subsystem
      settings: PortSchema="{\"entries\":[{\"content\":{\"headerSize\":26,\"margin\":15,\"minimumSpacing\":25,\"sides\":[{\"content\":{},\"type\":\"ConnectorPlacement.EquallySpacedRectSide\",\"uuid\":\"23792f18-2863-4199-9730-8799d4a474a5\"},{\"content\":{\"connectorIds\":[\"RConn1\",\"Out1\"],\"side\":\"RIGHT\"},\"type\":\"ConnectorPlacement.EquallySpacedRectSide\",\"uuid\":\"c8cda51b-7b41-45d2-a922-70343296893f\"},{\"content\":{\"side\":\"TOP\"},\"type\":\"ConnectorPlacement.EquallySpacedRectSide\",\"uuid\":\"3580f4a1-1924-4d7f-ad03-70e3a97c03ce\"}]},\"type\":\"ConnectorPlacement.EquallySpacedConnector\",\"uuid\":\"f1529067-176f-4d7b-82ef-d3d6162373fd\"}],\"packageUris\":[\"http://schema.mathworks.com/mf0/Connector/R2020b\"],\"version\":\"1.0\"}"
  Recovery state/health : Subsystem
      settings: PortSchema="{\"entries\":[{\"content\":{\"headerSize\":26,\"margin\":15,\"minimumSpacing\":25,\"sides\":[{\"content\":{\"connectorIds\":[\"In1\",\"In2\"]},\"type\":\"ConnectorPlacement.EquallySpacedRectSide\",\"uuid\":\"23792f18-2863-4199-9730-8799d4a474a5\"},{\"content\":{\"connectorIds\":[\"Out1\"],\"side\":\"RIGHT\"},\"type\":\"ConnectorPlacement.EquallySpacedRectSide\",\"uuid\":\"c8cda51b-7b41-45d2-a922-70343296893f\"},{\"content\":{\"side\":\"TOP\"},\"type\":\"ConnectorPlacement.EquallySpacedRectSide\",\"uuid\":\"3580f4a1-1924-4d7f-ad03-70e3a97c03ce\"}]},\"type\":\"ConnectorPlacement.EquallySpacedConnector\",\"uuid\":\"f1529067-176f-4d7b-82ef-d3d6162373fd\"}],\"packageUris\":[\"http://schema.mathworks.com/mf0/Connector/R2020b\"],\"version\":\"1.0\"}"
  IF-RLI-GND-01 : PMIOPort  Side=Right  ConnectionType=Bus: StructuralLoad
  IF-RLI-PRS-01 : PMIOPort  Port=2  Side=Right
  Bus Element Out1 : Outport  PortName=IF-RSM-SAF-01
  wires:
  Recovery mechanism/1(IF-RME-RSM-01) -> Recovery state/health/1(IF-RME-RSM-01)
  Recovery state/health/1(IF-RSM-SAF-01) -> Bus Element Out1/1
  Bus Element In1/1 -> Recovery state/health/2(IF-SAF-RSM-01)
  connections:
  Recovery mechanism/RConn1 -- Landing/catch load path/LConn1
  Landing/catch load path/RConn1 -- IF-RLI-GND-01/RConn1
  Landing/catch load path/RConn2 -- IF-RLI-PRS-01/RConn1

== system StarshipSystemModel/Starship/Structure and Mechanisms/Stage & Thrust Interfaces ==
  Hot-stage interface : Subsystem
      settings: PortSchema="{\"entries\":[{\"content\":{\"headerSize\":26,\"margin\":15,\"minimumSpacing\":25,\"sides\":[{\"content\":{},\"type\":\"ConnectorPlacement.EquallySpacedRectSide\",\"uuid\":\"23792f18-2863-4199-9730-8799d4a474a5\"},{\"content\":{\"connectorIds\":[\"RConn1\"],\"side\":\"RIGHT\"},\"type\":\"ConnectorPlacement.EquallySpacedRectSide\",\"uuid\":\"c8cda51b-7b41-45d2-a922-70343296893f\"},{\"content\":{\"side\":\"TOP\"},\"type\":\"ConnectorPlacement.EquallySpacedRectSide\",\"uuid\":\"3580f4a1-1924-4d7f-ad03-70e3a97c03ce\"}]},\"type\":\"ConnectorPlacement.EquallySpacedConnector\",\"uuid\":\"f1529067-176f-4d7b-82ef-d3d6162373fd\"}],\"packageUris\":[\"http://schema.mathworks.com/mf0/Connector/R2020b\"],\"version\":\"1.0\"}"
  Separation response : Subsystem
      settings: PortSchema="{\"entries\":[{\"content\":{\"headerSize\":26,\"margin\":15,\"minimumSpacing\":25,\"sides\":[{\"content\":{\"connectorIds\":[\"LConn1\"]},\"type\":\"ConnectorPlacement.EquallySpacedRectSide\",\"uuid\":\"23792f18-2863-4199-9730-8799d4a474a5\"},{\"content\":{\"connectorIds\":[\"RConn1\"],\"side\":\"RIGHT\"},\"type\":\"ConnectorPlacement.EquallySpacedRectSide\",\"uuid\":\"c8cda51b-7b41-45d2-a922-70343296893f\"},{\"content\":{\"side\":\"TOP\"},\"type\":\"ConnectorPlacement.EquallySpacedRectSide\",\"uuid\":\"3580f4a1-1924-4d7f-ad03-70e3a97c03ce\"}]},\"type\":\"ConnectorPlacement.EquallySpacedConnector\",\"uuid\":\"f1529067-176f-4d7b-82ef-d3d6162373fd\"}],\"packageUris\":[\"http://schema.mathworks.com/mf0/Connector/R2020b\"],\"version\":\"1.0\"}"
  Thrust-load introduction : Subsystem
      settings: PortSchema="{\"entries\":[{\"content\":{\"headerSize\":26,\"margin\":15,\"minimumSpacing\":25,\"sides\":[{\"content\":{\"connectorIds\":[\"RConn1\",\"RConn2\"]},\"type\":\"ConnectorPlacement.EquallySpacedRectSide\",\"uuid\":\"23792f18-2863-4199-9730-8799d4a474a5\"},{\"content\":{\"connectorIds\":[\"RConn3\"],\"side\":\"RIGHT\"},\"type\":\"ConnectorPlacement.EquallySpacedRectSide\",\"uuid\":\"c8cda51b-7b41-45d2-a922-70343296893f\"},{\"content\":{\"side\":\"TOP\"},\"type\":\"ConnectorPlacement.EquallySpacedRectSide\",\"uuid\":\"3580f4a1-1924-4d7f-ad03-70e3a97c03ce\"}]},\"type\":\"ConnectorPlacement.EquallySpacedConnector\",\"uuid\":\"f1529067-176f-4d7b-82ef-d3d6162373fd\"}],\"packageUris\":[\"http://schema.mathworks.com/mf0/Connector/R2020b\"],\"version\":\"1.0\"}"
  IF-BMT-TLI-01 : PMIOPort  Side=Right  ConnectionType=Bus: StructuralLoad
  IF-SMT-TLI-01 : PMIOPort  Port=2  Side=Right  ConnectionType=Bus: StructuralLoad
  IF-TLI-LDT-01 : PMIOPort  Port=3  Side=Right
  IF-SLS-LDT-01 : PMIOPort  Port=4  Side=Right
  connections:
  Thrust-load introduction/RConn3 -- IF-TLI-LDT-01/RConn1
  Hot-stage interface/RConn1 -- Separation response/LConn1
  Thrust-load introduction/RConn1 -- IF-BMT-TLI-01/RConn1
  Thrust-load introduction/RConn2 -- IF-SMT-TLI-01/RConn1
  Separation response/RConn1 -- IF-SLS-LDT-01/RConn1

== system StarshipSystemModel/Starship/Thermal Protection/Ship Primary TPS ==
  Bus Element In2 : Inport  PortName=IF-SNZ-STP-01
  Bus Element In1 : Inport  Port=2  PortName=IF-ATM-STP-01
  Base heat-shield region : Subsystem
      settings: PortSchema="{\"entries\":[{\"content\":{\"headerSize\":26,\"margin\":15,\"minimumSpacing\":25,\"sides\":[{\"content\":{},\"type\":\"ConnectorPlacement.EquallySpacedRectSide\",\"uuid\":\"e0cfb70a-2480-46ad-8838-78efdb61b60e\"},{\"content\":{\"side\":\"RIGHT\"},\"type\":\"ConnectorPlacement.EquallySpacedRectSide\",\"uuid\":\"0844e172-3ed8-42bd-94dc-a51d08e37039\"},{\"content\":{\"side\":\"TOP\"},\"type\":\"ConnectorPlacement.EquallySpacedRectSide\",\"uuid\":\"2415ea6e-ae7d-422f-a1cc-5a10cd0c87f7\"}]},\"type\":\"ConnectorPlacement.EquallySpacedConnector\",\"uuid\":\"814347a2-9201-4b2d-b96f-a93fca4a3c45\"}],\"packageUris\":[\"http://schema.mathworks.com/mf0/Connector/R2020b\"],\"version\":\"1.0\"}"
  Control-surface thermal protection : Subsystem
      settings: PortSchema="{\"entries\":[{\"content\":{\"headerSize\":26,\"margin\":15,\"minimumSpacing\":25,\"sides\":[{\"content\":{},\"type\":\"ConnectorPlacement.EquallySpacedRectSide\",\"uuid\":\"e0cfb70a-2480-46ad-8838-78efdb61b60e\"},{\"content\":{\"connectorIds\":[\"Out1\"],\"side\":\"RIGHT\"},\"type\":\"ConnectorPlacement.EquallySpacedRectSide\",\"uuid\":\"0844e172-3ed8-42bd-94dc-a51d08e37039\"},{\"content\":{\"side\":\"TOP\"},\"type\":\"ConnectorPlacement.EquallySpacedRectSide\",\"uuid\":\"2415ea6e-ae7d-422f-a1cc-5a10cd0c87f7\"}]},\"type\":\"ConnectorPlacement.EquallySpacedConnector\",\"uuid\":\"814347a2-9201-4b2d-b96f-a93fca4a3c45\"}],\"packageUris\":[\"http://schema.mathworks.com/mf0/Connector/R2020b\"],\"version\":\"1.0\"}"
  Localized high-heating protection : Subsystem
      settings: PortSchema="{\"entries\":[{\"content\":{\"headerSize\":26,\"margin\":15,\"minimumSpacing\":25,\"sides\":[{\"content\":{},\"type\":\"ConnectorPlacement.EquallySpacedRectSide\",\"uuid\":\"e0cfb70a-2480-46ad-8838-78efdb61b60e\"},{\"content\":{\"connectorIds\":[\"Out1\"],\"side\":\"RIGHT\"},\"type\":\"ConnectorPlacement.EquallySpacedRectSide\",\"uuid\":\"0844e172-3ed8-42bd-94dc-a51d08e37039\"},{\"content\":{\"side\":\"TOP\"},\"type\":\"ConnectorPlacement.EquallySpacedRectSide\",\"uuid\":\"2415ea6e-ae7d-422f-a1cc-5a10cd0c87f7\"}]},\"type\":\"ConnectorPlacement.EquallySpacedConnector\",\"uuid\":\"814347a2-9201-4b2d-b96f-a93fca4a3c45\"}],\"packageUris\":[\"http://schema.mathworks.com/mf0/Connector/R2020b\"],\"version\":\"1.0\"}"
  Primary TPS acreage / tile field : Subsystem
      settings: PortSchema="{\"entries\":[{\"content\":{\"headerSize\":26,\"margin\":15,\"minimumSpacing\":25,\"sides\":[{\"content\":{\"connectorIds\":[\"In1\",\"In2\"]},\"type\":\"ConnectorPlacement.EquallySpacedRectSide\",\"uuid\":\"e0cfb70a-2480-46ad-8838-78efdb61b60e\"},{\"content\":{\"connectorIds\":[\"Out1\",\"RConn1\"],\"side\":\"RIGHT\"},\"type\":\"ConnectorPlacement.EquallySpacedRectSide\",\"uuid\":\"0844e172-3ed8-42bd-94dc-a51d08e37039\"},{\"content\":{\"side\":\"TOP\"},\"type\":\"ConnectorPlacement.EquallySpacedRectSide\",\"uuid\":\"2415ea6e-ae7d-422f-a1cc-5a10cd0c87f7\"}]},\"type\":\"ConnectorPlacement.EquallySpacedConnector\",\"uuid\":\"814347a2-9201-4b2d-b96f-a93fca4a3c45\"}],\"packageUris\":[\"http://schema.mathworks.com/mf0/Connector/R2020b\"],\"version\":\"1.0\"}"
  IF-STP-PRS-01 : PMIOPort  Side=Right  ConnectionType=Bus: ThermalNetwork
  Bus Element Out2 : Outport  PortName=IF-STP-ACR-TBI-GAP-01
  Bus Element Out3 : Outport  Port=2  PortName=IF-STP-CTL-TBI-CTL-01
  Bus Element Out4 : Outport  Port=3  PortName=IF-STP-LOC-TBI-STP-01
  wires:
  Primary TPS acreage / tile field/1(IF-STP-ACR-TBI-GAP-01) -> Bus Element Out2/1
  Control-surface thermal protection/1(IF-STP-CTL-TBI-CTL-01) -> Bus Element Out3/1
  Localized high-heating protection/1(IF-STP-LOC-TBI-STP-01) -> Bus Element Out4/1
  Bus Element In1/1 -> Primary TPS acreage / tile field/1(IF-ATM-STP-01)
  Bus Element In2/1 -> Primary TPS acreage / tile field/2(IF-SNZ-STP-01)
  connections:
  Primary TPS acreage / tile field/RConn1 -- IF-STP-PRS-01/RConn1

== system StarshipSystemModel/Starship/Thermal Protection/Super Heavy Thermal Protection ==
  Bus Element In2 : Inport  PortName=IF-BNZ-BTP-01
  Bus Element In1 : Inport  Port=2  PortName=IF-ATM-BTP-01
  Base heat-shield region : Subsystem
      settings: PortSchema="{\"entries\":[{\"content\":{\"headerSize\":26,\"margin\":15,\"minimumSpacing\":25,\"sides\":[{\"content\":{},\"type\":\"ConnectorPlacement.EquallySpacedRectSide\",\"uuid\":\"e0cfb70a-2480-46ad-8838-78efdb61b60e\"},{\"content\":{\"side\":\"RIGHT\"},\"type\":\"ConnectorPlacement.EquallySpacedRectSide\",\"uuid\":\"0844e172-3ed8-42bd-94dc-a51d08e37039\"},{\"content\":{\"side\":\"TOP\"},\"type\":\"ConnectorPlacement.EquallySpacedRectSide\",\"uuid\":\"2415ea6e-ae7d-422f-a1cc-5a10cd0c87f7\"}]},\"type\":\"ConnectorPlacement.EquallySpacedConnector\",\"uuid\":\"814347a2-9201-4b2d-b96f-a93fca4a3c45\"}],\"packageUris\":[\"http://schema.mathworks.com/mf0/Connector/R2020b\"],\"version\":\"1.0\"}"
  Forward heat-shield / interstage : Subsystem
      settings: PortSchema="{\"entries\":[{\"content\":{\"headerSize\":26,\"margin\":15,\"minimumSpacing\":25,\"sides\":[{\"content\":{},\"type\":\"ConnectorPlacement.EquallySpacedRectSide\",\"uuid\":\"e0cfb70a-2480-46ad-8838-78efdb61b60e\"},{\"content\":{\"connectorIds\":[\"Out1\"],\"side\":\"RIGHT\"},\"type\":\"ConnectorPlacement.EquallySpacedRectSide\",\"uuid\":\"0844e172-3ed8-42bd-94dc-a51d08e37039\"},{\"content\":{\"side\":\"TOP\"},\"type\":\"ConnectorPlacement.EquallySpacedRectSide\",\"uuid\":\"2415ea6e-ae7d-422f-a1cc-5a10cd0c87f7\"}]},\"type\":\"ConnectorPlacement.EquallySpacedConnector\",\"uuid\":\"814347a2-9201-4b2d-b96f-a93fca4a3c45\"}],\"packageUris\":[\"http://schema.mathworks.com/mf0/Connector/R2020b\"],\"version\":\"1.0\"}"
  Localized thermal protection : Subsystem
      settings: PortSchema="{\"entries\":[{\"content\":{\"headerSize\":26,\"margin\":15,\"minimumSpacing\":25,\"sides\":[{\"content\":{},\"type\":\"ConnectorPlacement.EquallySpacedRectSide\",\"uuid\":\"e0cfb70a-2480-46ad-8838-78efdb61b60e\"},{\"content\":{\"connectorIds\":[\"RConn1\",\"Out1\"],\"side\":\"RIGHT\"},\"type\":\"ConnectorPlacement.EquallySpacedRectSide\",\"uuid\":\"0844e172-3ed8-42bd-94dc-a51d08e37039\"},{\"content\":{\"side\":\"TOP\"},\"type\":\"ConnectorPlacement.EquallySpacedRectSide\",\"uuid\":\"2415ea6e-ae7d-422f-a1cc-5a10cd0c87f7\"}]},\"type\":\"ConnectorPlacement.EquallySpacedConnector\",\"uuid\":\"814347a2-9201-4b2d-b96f-a93fca4a3c45\"}],\"packageUris\":[\"http://schema.mathworks.com/mf0/Connector/R2020b\"],\"version\":\"1.0\"}"
  Primary TPS acreage : Subsystem
      settings: PortSchema="{\"entries\":[{\"content\":{\"headerSize\":26,\"margin\":15,\"minimumSpacing\":25,\"sides\":[{\"content\":{\"connectorIds\":[\"In1\",\"In2\"]},\"type\":\"ConnectorPlacement.EquallySpacedRectSide\",\"uuid\":\"e0cfb70a-2480-46ad-8838-78efdb61b60e\"},{\"content\":{\"connectorIds\":[\"Out1\"],\"side\":\"RIGHT\"},\"type\":\"ConnectorPlacement.EquallySpacedRectSide\",\"uuid\":\"0844e172-3ed8-42bd-94dc-a51d08e37039\"},{\"content\":{\"side\":\"TOP\"},\"type\":\"ConnectorPlacement.EquallySpacedRectSide\",\"uuid\":\"2415ea6e-ae7d-422f-a1cc-5a10cd0c87f7\"}]},\"type\":\"ConnectorPlacement.EquallySpacedConnector\",\"uuid\":\"814347a2-9201-4b2d-b96f-a93fca4a3c45\"}],\"packageUris\":[\"http://schema.mathworks.com/mf0/Connector/R2020b\"],\"version\":\"1.0\"}"
  IF-BTP-PRS-01 : PMIOPort  Side=Right  ConnectionType=Bus: ThermalNetwork
  Bus Element Out2 : Outport  PortName=IF-BTP-ACR-TBI-GAP-01
  Bus Element Out3 : Outport  Port=2  PortName=IF-BTP-FHI-TBI-INT-01
  Bus Element Out4 : Outport  Port=3  PortName=IF-BTP-LOC-TBI-STP-01
  wires:
  Primary TPS acreage/1(IF-BTP-ACR-TBI-GAP-01) -> Bus Element Out2/1
  Forward heat-shield / interstage/1(IF-BTP-FHI-TBI-INT-01) -> Bus Element Out3/1
  Localized thermal protection/1(IF-BTP-LOC-TBI-STP-01) -> Bus Element Out4/1
  Bus Element In2/1 -> Primary TPS acreage/1(IF-BNZ-BTP-01)
  Bus Element In1/1 -> Primary TPS acreage/2(IF-ATM-BTP-01)
  connections:
  Localized thermal protection/RConn1 -- IF-BTP-PRS-01/RConn1
